simulink model "lab3_q1"  (R2026b)
settings: Solver=FixedStepAuto  StopTime=40  FixedStep=0.001
model workspace (MAT data in the model file):
  k_1 = -1.81
  tau = 0.0231
settings Model: Creator=erica  LastModifiedBy=lucasadesky

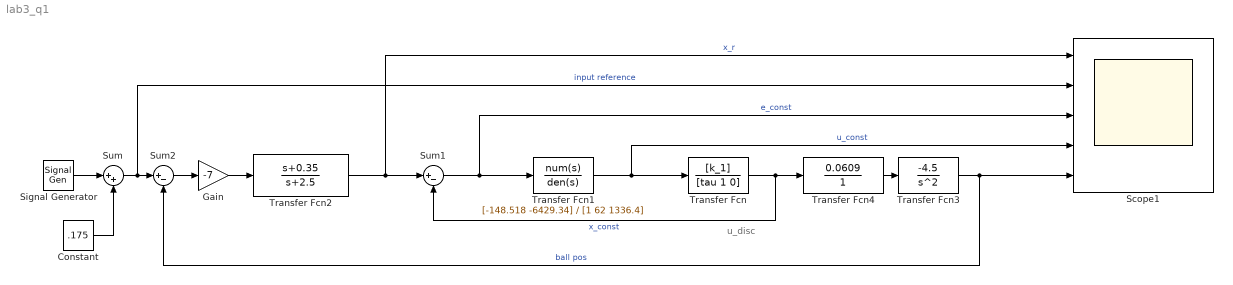
== system lab3_q1 ==
  note: u_disc
  Constant : Constant  Value=.175
  Gain : Gain  Gain=-7
  Scope1 : Scope  NumInputPorts=5
      settings: ActiveDisplayYMinimum=-1.1617696944011375  ActiveDisplayYMaximum=1.5533881628228481
  Signal Generator : SignalGenerator  WaveForm=square  Amplitude=.075  Frequency=1/20
  Sum : Sum  Inputs=|++
  Sum1 : Sum  Inputs=|+-
  Sum2 : Sum  Inputs=|+-
  Transfer Fcn : TransferFcn  Numerator=[k_1]  Denominator=[tau 1 0]
  Transfer Fcn1 : TransferFcn  Numerator=[-148.518 -6429.34]  Denominator=[1 62 1336.4]
  Transfer Fcn2 : TransferFcn  Numerator=[1 0.35]  Denominator=[1 2.5]
  Transfer Fcn3 : TransferFcn  Numerator=[-4.5]  Denominator=[1 0 0]
  Transfer Fcn4 : TransferFcn  Numerator=0.0609  Denominator=[1]
  wires:
  Transfer Fcn1/1 -> Scope1/4, Transfer Fcn/1  "u_const"
  Transfer Fcn/1 -> Transfer Fcn4/1, Sum1/2  "x_const"
  Transfer Fcn2/1 -> Scope1/1, Sum1/1  "x_r"
  Sum1/1 -> Scope1/3, Transfer Fcn1/1  "e_const"
  Gain/1 -> Transfer Fcn2/1
  Signal Generator/1 -> Sum/1
  Constant/1 -> Sum/2
  Sum2/1 -> Gain/1
  Transfer Fcn3/1 -> Scope1/5, Sum2/2  "ball pos"
  Transfer Fcn4/1 -> Transfer Fcn3/1
  Sum/1 -> Scope1/2, Sum2/1  "input reference"
